simulink model "Compensated_FOC"  (R2023a)
settings: Solver=FixedStepDiscrete  StartTime=0.0  StopTime=SC.T  FixedStep=P.dt  RelTol=1e-3
PreLoadFcn:
  | d_ = fileparts(get_param(bdroot,'FileName')); addpath(d_, fullfile(d_, '..', 'Common')); clear d_; comp_foc_init;
values from neighbouring files (symbols this model uses):
  DECIM = 10    [comp_foc_init.m]
  P = bldc_params()    [comp_foc_init.m]
  TAB = struct()    [comp_foc_init.m]
  TAB_SHIFT = 0    [comp_foc_calib.mat]    (also in comp_foc_init.m; run_comp_foc.m = shv(bs))
  THETA_OFF = -1.57079632679    [comp_foc_calib.mat]    (also in comp_foc_init.m)
libraries: bldc_plant_lib x6, slpidlib x3, spspowerguiLib x1
settings Model: Creator=PC  LastModifiedBy=PC

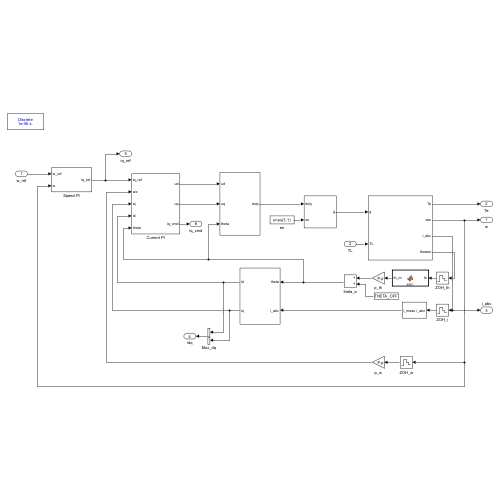
[thumbnail: Simulink's stored preview of the top-level diagram]
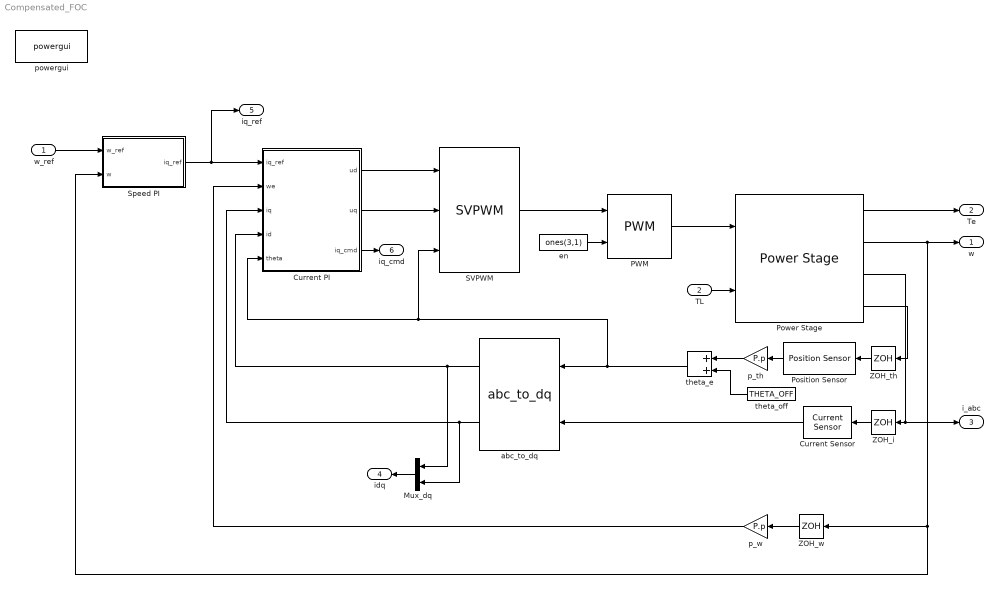
== system Compensated_FOC ==
  w_ref : Inport  Interpolate=off
  TL : Inport  Port=2  Interpolate=off
  Current PI : Subsystem
  Current Sensor : bldc_plant_lib/Current Sensor  Description=Phase-current sensors: i_meas = P.CS.M*(P.CS.gain.*i_abc + P.CS.off). Ideal by default (bldc_set_sensor).  SystemSampleTime=-1  VariantActivationTime=update diagram  Latency=0  AutoFrameSizeCalculation=off
  Mux_dq : Mux  Inputs=2
  PWM : bldc_plant_lib/PWM  SystemSampleTime=-1  VariantActivationTime=update diagram  Latency=0  AutoFrameSizeCalculation=off
  Position Sensor : bldc_plant_lib/Position Sensor  Description=Position sensor: quantized mechanical angle + mounting offset (P.ENC, bldc_set_encoder). Ideal by default.  SystemSampleTime=-1  VariantActivationTime=update diagram  Latency=0  AutoFrameSizeCalculation=off
      settings: LibrarySourceBlock=|
      | simulink/User-Defined
      | Functions/MATLAB Function
  Power Stage : bldc_plant_lib/Power Stage  SystemSampleTime=-1  VariantActivationTime=update diagram  Latency=0  AutoFrameSizeCalculation=off
  SVPWM : bldc_plant_lib/SVPWM  SystemSampleTime=-1  VariantActivationTime=update diagram  Latency=0  AutoFrameSizeCalculation=off
  Speed PI : Subsystem
  ZOH_i : ZeroOrderHold  SampleTime=P.Ts
  ZOH_th : ZeroOrderHold  SampleTime=P.Ts
  ZOH_w : ZeroOrderHold  SampleTime=P.Ts
  abc_to_dq : bldc_plant_lib/abc_to_dq  SystemSampleTime=-1  VariantActivationTime=update diagram  Latency=0  AutoFrameSizeCalculation=off
  en : Constant  Value=ones(3,1)
  p_th : Gain  Gain=P.p
  p_w : Gain  Gain=P.p
  powergui : spspowerguiLib/powergui  Priority=1  SimulationMode=Discrete  SampleTime=P.dt  frequency=60  Iterations=50  frequencyindice=0  Pbase=100e6  ErrMax=1e-4  UnitsV=kV  UnitsW=MW  buscounter=0  FunctionMessages=off  echomessages=off  EnableUseOfTLC=off  CurrentSourceSwitches=off  DisableSnubberDevices=off  DisableRonSwitches=off  DisableVfSwitches=off  DisplayEquations=off  AutomaticDiscreteSolvers=off  SolverType=Tustin/Backward Euler (TBE)  Interpol=off  ExternalGateDelay=off  methode=off  Ts=100  x0status=blocks  SPID=on  SwTol=0  HookPort=off  NonlinearTolerance=1e-4  nMaxIteration=100  ContinueOnMaxIteration=off  RestoreLinks=warning  ResistiveCurrentMeasurement=off  Frange=[0:2:500]  Ylog=off  Xlog=on  ShowGrid=off  save=off  variable=ZData  structure=0  ZoomFFT=off  StartTime=0.0  cycles=1  DisplayStyle=1  fundamental=60  FreqAxis=off  MaxFrequency=1000  frequencyindicesteady=1  RmsSteady=1  display=off
  theta_e : Sum
  theta_off : Constant  Value=THETA_OFF
  w : Outport  SampleTime=DECIM*P.dt
  Te : Outport  Port=2  SampleTime=DECIM*P.dt
  i_abc : Outport  Port=3  SampleTime=DECIM*P.dt
  idq : Outport  Port=4
  iq_ref : Outport  Port=5
  iq_cmd : Outport  Port=6
  wires:
  w_ref/1 -> Speed PI/1(w_ref)
  Speed PI/1(iq_ref) -> Current PI/1(iq_ref), iq_ref/1
  Current PI/1(ud) -> SVPWM/1
  Current PI/2(uq) -> SVPWM/2
  Current PI/3(iq_cmd) -> iq_cmd/1
  SVPWM/1 -> PWM/1
  en/1 -> PWM/2
  PWM/1 -> Power Stage/1
  TL/1 -> Power Stage/2
  Power Stage/1 -> Te/1
  Power Stage/2 -> ZOH_w/1, Speed PI/2(w), w/1
  Power Stage/3 -> ZOH_i/1, i_abc/1
  Power Stage/4 -> ZOH_th/1
  p_th/1 -> theta_e/1
  theta_off/1 -> theta_e/2
  theta_e/1 -> abc_to_dq/1, Current PI/5(theta), SVPWM/3
  abc_to_dq/1 -> Current PI/4(id), Mux_dq/1
  abc_to_dq/2 -> Current PI/3(iq), Mux_dq/2
  Mux_dq/1 -> idq/1
  ZOH_w/1 -> p_w/1
  p_w/1 -> Current PI/2(we)
  ZOH_i/1 -> Current Sensor/1
  Current Sensor/1 -> abc_to_dq/2
  ZOH_th/1 -> Position Sensor/1
  Position Sensor/1 -> p_th/1

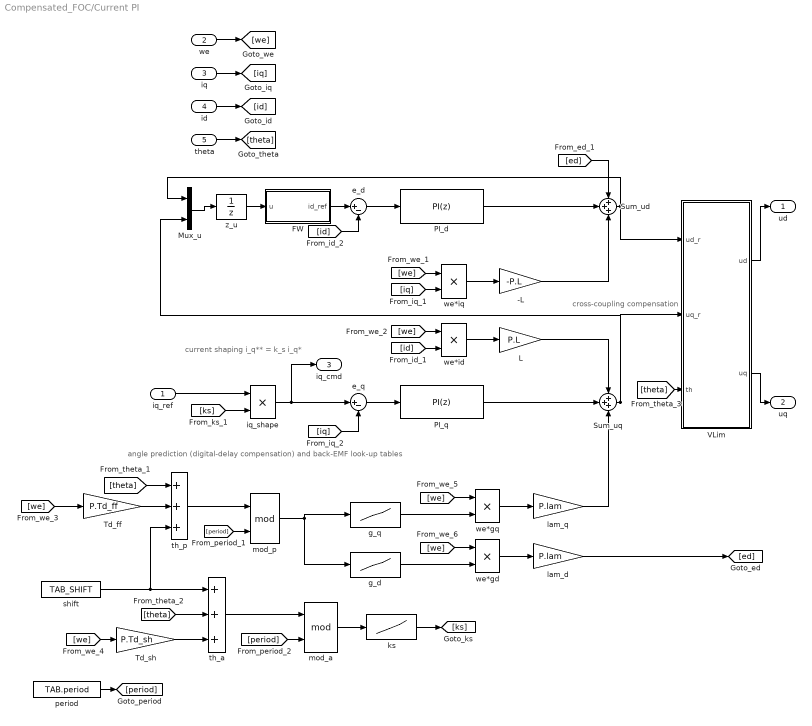
== system Compensated_FOC/Current PI ==
  note: cross-coupling compensation
  note: angle prediction (digital-delay compensation) and back-EMF look-up tables
  note: current shaping i_q** = k_s i_q*
  iq_ref : Inport
  we : Inport  Port=2
  iq : Inport  Port=3
  id : Inport  Port=4
  theta : Inport  Port=5
  -L : Gain  Gain=-P.L
  FW : MATLAB Function  TreatAsAtomicUnit=on  SystemSampleTime=P.Ts
  L : Gain  Gain=P.L
  Mux_u : Mux  Inputs=2
  PI_d : slpidlib/PID Controller  Controller=PI  Form=Parallel  TimeDomain=Discrete-time  UseExternalTs=off  SampleTime=P.Ts  IntegratorMethod=Forward Euler  FilterMethod=Forward Euler  ControllerParametersSource=internal  P=P.Kp_i  I=P.Ki_i  UseKiTs=off  D=0  N=100  UseFilter=on  TunerSelectOption=Transfer Function Based (PID Tuner App)  InitialConditionSource=internal  InitialConditionForIntegrator=0  InitialConditionForFilter=0  DifferentiatorICPrevScaledInput=0  ExternalReset=none  TrackingMode=off  Kt=1  LimitOutput=on  SatLimitsSource=internal  UpperSaturationLimit=P.Vm  LowerSaturationLimit=-P.Vm  LinearizeAsGain=off  AntiWindupMode=back-calculation  Kb=(P.Ki_i)/(P.Kp_i)  LimitIntegrator=off  UpperIntegratorSaturationLimit=inf  LowerIntegratorSaturationLimit=-inf  POutMin=[]  POutMax=[]  IOutMin=[]  IOutMax=[]  DOutMin=[]  DOutMax=[]  NOutMin=[]  NOutMax=[]  SumOutMin=[]  SumOutMax=[]  SaturationOutMin=[]  SaturationOutMax=[]  PParamMin=[]  PParamMax=[]  IParamMin=[]  IParamMax=[]  DParamMin=[]  DParamMax=[]  NParamMin=[]  NParamMax=[]  KbParamMin=[]  KbParamMax=[]  KtParamMin=[]  KtParamMax=[]  KbOutMin=[]  KbOutMax=[]  KtOutMin=[]  KtOutMax=[]  IntegratorOutMin=[]  IntegratorOutMax=[]  FilterOutMin=[]  FilterOutMax=[]  SumI1OutMin=[]  SumI1OutMax=[]  SumI2OutMin=[]  SumI2OutMax=[]  SumI3OutMin=[]  SumI3OutMax=[]  SumI4OutMin=[]  SumI4OutMax=[]  SumDOutMin=[]  SumDOutMax=[]  DifferentiatorOutMin=[]  DifferentiatorOutMax=[]  FilterDiffOutCoefMin=[]  FilterDiffOutCoefMax=[]  ReciprocalOutMin=[]  ReciprocalOutMax=[]  SumDenOutMin=[]  SumDenOutMax=[]  SumNumOutMin=[]  SumNumOutMax=[]  DivideOutMin=[]  DivideOutMax=[]  UdiffTsProdOutMin=[]  UdiffTsProdOutMax=[]  NTsProdOutMin=[]  NTsProdOutMax=[]  UintegralTsProdOutMin=[]  UintegralTsProdOutMax=[]  UngainTsProdOutMin=[]  UngainTsProdOutMax=[]  ClampingZeroOutDataTypeStr=Inherit: Inherit via back propagation  ClampingZeroOutMin=[]  ClampingZeroOutMax=[]  FilterDenConstantOutDataTypeStr=Inherit: Inherit via back propagation  FilterDenConstantOutMin=[]  FilterDenConstantOutMax=[]  PCopyOutDataTypeStr=Inherit: Inherit via back propagation  PCopyOutMin=[]  PCopyOutMax=[]  NCopyOutDataTypeStr=Inherit: Inherit via back propagation  NCopyOutMin=[]  NCopyOutMax=[]  IntegratorContinuousStateAttributes=''  IntegratorStateMustResolveToSignalObject=off  IntegratorRTWStateStorageClass=Auto  FilterContinuousStateAttributes=''  FilterStateMustResolveToSignalObject=off  FilterRTWStateStorageClass=Auto  ParallelPVariant=InternalParameters  IdealPVariant=Disabled  IVariant=InternalParameters  DVariant=Disabled  IntegratorVariant=Discrete  SatVariant=Enabled  AWVariant=BackCalculation  PCopyVariant=Disabled  TRVariant=Disabled  FdbkBlocksVariant=Forward  IdealPFdbkVariant=Disabled  SatFdbkVariant=Disabled  DerivativeFilterVariant=Disabled  NVariant=Disabled  NCopyVariant=Disabled_SignalSpec  FilterICVariant=Disabled  IntegratorICVariant=InternalICs  ExternalResetVariant=Disabled  TRSumVariant=Passthrough  SumFdbkVariant=Disabled  SumVariant=Sum_PI  TsampFilterVariant=InternalTs  TsampNgainVariant=Passthrough  TsampIntegralVariant=Disabled_SignalSpec  ExternalSaturationOutDataTypeStr=Inherit: Same as second input
      settings: LibrarySourceBlock=simulink/Discrete/Discrete PID Controller
  PI_q : slpidlib/PID Controller  Controller=PI  Form=Parallel  TimeDomain=Discrete-time  UseExternalTs=off  SampleTime=P.Ts  IntegratorMethod=Forward Euler  FilterMethod=Forward Euler  ControllerParametersSource=internal  P=P.Kp_i  I=P.Ki_i  UseKiTs=off  D=0  N=100  UseFilter=on  TunerSelectOption=Transfer Function Based (PID Tuner App)  InitialConditionSource=internal  InitialConditionForIntegrator=0  InitialConditionForFilter=0  DifferentiatorICPrevScaledInput=0  ExternalReset=none  TrackingMode=off  Kt=1  LimitOutput=on  SatLimitsSource=internal  UpperSaturationLimit=P.Vm  LowerSaturationLimit=-P.Vm  LinearizeAsGain=off  AntiWindupMode=back-calculation  Kb=(P.Ki_i)/(P.Kp_i)  LimitIntegrator=off  UpperIntegratorSaturationLimit=inf  LowerIntegratorSaturationLimit=-inf  POutMin=[]  POutMax=[]  IOutMin=[]  IOutMax=[]  DOutMin=[]  DOutMax=[]  NOutMin=[]  NOutMax=[]  SumOutMin=[]  SumOutMax=[]  SaturationOutMin=[]  SaturationOutMax=[]  PParamMin=[]  PParamMax=[]  IParamMin=[]  IParamMax=[]  DParamMin=[]  DParamMax=[]  NParamMin=[]  NParamMax=[]  KbParamMin=[]  KbParamMax=[]  KtParamMin=[]  KtParamMax=[]  KbOutMin=[]  KbOutMax=[]  KtOutMin=[]  KtOutMax=[]  IntegratorOutMin=[]  IntegratorOutMax=[]  FilterOutMin=[]  FilterOutMax=[]  SumI1OutMin=[]  SumI1OutMax=[]  SumI2OutMin=[]  SumI2OutMax=[]  SumI3OutMin=[]  SumI3OutMax=[]  SumI4OutMin=[]  SumI4OutMax=[]  SumDOutMin=[]  SumDOutMax=[]  DifferentiatorOutMin=[]  DifferentiatorOutMax=[]  FilterDiffOutCoefMin=[]  FilterDiffOutCoefMax=[]  ReciprocalOutMin=[]  ReciprocalOutMax=[]  SumDenOutMin=[]  SumDenOutMax=[]  SumNumOutMin=[]  SumNumOutMax=[]  DivideOutMin=[]  DivideOutMax=[]  UdiffTsProdOutMin=[]  UdiffTsProdOutMax=[]  NTsProdOutMin=[]  NTsProdOutMax=[]  UintegralTsProdOutMin=[]  UintegralTsProdOutMax=[]  UngainTsProdOutMin=[]  UngainTsProdOutMax=[]  ClampingZeroOutDataTypeStr=Inherit: Inherit via back propagation  ClampingZeroOutMin=[]  ClampingZeroOutMax=[]  FilterDenConstantOutDataTypeStr=Inherit: Inherit via back propagation  FilterDenConstantOutMin=[]  FilterDenConstantOutMax=[]  PCopyOutDataTypeStr=Inherit: Inherit via back propagation  PCopyOutMin=[]  PCopyOutMax=[]  NCopyOutDataTypeStr=Inherit: Inherit via back propagation  NCopyOutMin=[]  NCopyOutMax=[]  IntegratorContinuousStateAttributes=''  IntegratorStateMustResolveToSignalObject=off  IntegratorRTWStateStorageClass=Auto  FilterContinuousStateAttributes=''  FilterStateMustResolveToSignalObject=off  FilterRTWStateStorageClass=Auto  ParallelPVariant=InternalParameters  IdealPVariant=Disabled  IVariant=InternalParameters  DVariant=Disabled  IntegratorVariant=Discrete  SatVariant=Enabled  AWVariant=BackCalculation  PCopyVariant=Disabled  TRVariant=Disabled  FdbkBlocksVariant=Forward  IdealPFdbkVariant=Disabled  SatFdbkVariant=Disabled  DerivativeFilterVariant=Disabled  NVariant=Disabled  NCopyVariant=Disabled_SignalSpec  FilterICVariant=Disabled  IntegratorICVariant=InternalICs  ExternalResetVariant=Disabled  TRSumVariant=Passthrough  SumFdbkVariant=Disabled  SumVariant=Sum_PI  TsampFilterVariant=InternalTs  TsampNgainVariant=Passthrough  TsampIntegralVariant=Disabled_SignalSpec  ExternalSaturationOutDataTypeStr=Inherit: Same as second input
      settings: LibrarySourceBlock=simulink/Discrete/Discrete PID Controller
  Sum_ud : Sum  Inputs=+++
  Sum_uq : Sum  Inputs=+++
  Td_ff : Gain  Gain=P.Td_ff
  Td_sh : Gain  Gain=P.Td_sh
  VLim : MATLAB Function  TreatAsAtomicUnit=on  SystemSampleTime=P.Ts
  e_d : Sum  Inputs=|+-
  e_q : Sum  Inputs=|+-
  g_d : Lookup_n-D  NumberOfTableDimensions=1  BreakpointsForDimension1=TAB.th  Table=TAB.gd  ExtrapMethod=Clip  InternalRulePriority=Speed  RndMeth=Simplest
  g_q : Lookup_n-D  NumberOfTableDimensions=1  BreakpointsForDimension1=TAB.th  Table=TAB.gq  ExtrapMethod=Clip  InternalRulePriority=Speed  RndMeth=Simplest
  iq_shape : Product
  ks : Lookup_n-D  NumberOfTableDimensions=1  BreakpointsForDimension1=TAB.th  Table=TAB.ks  ExtrapMethod=Clip  InternalRulePriority=Speed  RndMeth=Simplest
  lam_d : Gain  Gain=P.lam
  lam_q : Gain  Gain=P.lam
  mod_a : Math  Operator=mod
  mod_p : Math  Operator=mod
  period : Constant  Value=TAB.period
  shift : Constant  Value=TAB_SHIFT
  th_a : Sum  Inputs=+++
  th_p : Sum  Inputs=+++
  we*gd : Product
  we*gq : Product
  we*id : Product
  we*iq : Product
  z_u : UnitDelay  InitialCondition=[0;0]  SampleTime=P.Ts
  ud : Outport
  uq : Outport  Port=2
  iq_cmd : Outport  Port=3
  wires:
  we/1 -> [we]
  [we] -> we*iq/1
  [we] -> we*id/1
  [we] -> Td_ff/1
  [we] -> Td_sh/1
  [we] -> we*gq/1
  [we] -> we*gd/1
  iq/1 -> [iq]
  [iq] -> we*iq/2
  [iq] -> e_q/2
  id/1 -> [id]
  [id] -> we*id/2
  [id] -> e_d/2
  theta/1 -> [theta]
  [theta] -> th_p/1
  [theta] -> th_a/2
  lam_d/1 -> [ed]
  [ed] -> Sum_ud/1
  period/1 -> [period]
  [period] -> mod_p/2
  [period] -> mod_a/2
  ks/1 -> [ks]
  [ks] -> iq_shape/2
  -L/1 -> Sum_ud/3
  L/1 -> Sum_uq/1
  PI_d/1 -> Sum_ud/2
  PI_q/1 -> Sum_uq/2
  Td_ff/1 -> th_p/2
  Td_sh/1 -> th_a/3
  e_d/1 -> PI_d/1
  e_q/1 -> PI_q/1
  g_d/1 -> we*gd/2
  g_q/1 -> we*gq/2
  iq_ref/1 -> iq_shape/1
  iq_shape/1 -> e_q/1, iq_cmd/1
  lam_q/1 -> Sum_uq/3
  mod_a/1 -> ks/1
  mod_p/1 -> g_d/1, g_q/1
  shift/1 -> th_p/3, th_a/1
  th_a/1 -> mod_a/1
  th_p/1 -> mod_p/1
  we*gd/1 -> lam_d/1
  we*gq/1 -> lam_q/1
  we*id/1 -> L/1
  we*iq/1 -> -L/1
  Sum_ud/1 -> VLim/1(ud_r), Mux_u/1
  Sum_uq/1 -> VLim/2(uq_r), Mux_u/2
  [theta] -> VLim/3(th)
  VLim/1(ud) -> ud/1
  VLim/2(uq) -> uq/1
  Mux_u/1 -> z_u/1
  z_u/1 -> FW/1(u)
  FW/1(id_ref) -> e_d/1

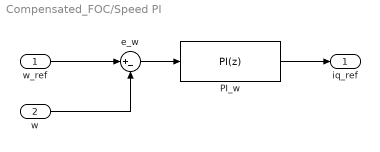
== system Compensated_FOC/Speed PI ==
  w_ref : Inport
  w : Inport  Port=2
  PI_w : slpidlib/PID Controller  Controller=PI  Form=Parallel  TimeDomain=Discrete-time  UseExternalTs=off  SampleTime=P.Tsw  IntegratorMethod=Forward Euler  FilterMethod=Forward Euler  ControllerParametersSource=internal  P=P.Kp_w_foc  I=P.Ki_w_foc  UseKiTs=off  D=0  N=100  UseFilter=on  TunerSelectOption=Transfer Function Based (PID Tuner App)  InitialConditionSource=internal  InitialConditionForIntegrator=0  InitialConditionForFilter=0  DifferentiatorICPrevScaledInput=0  ExternalReset=none  TrackingMode=off  Kt=1  LimitOutput=on  SatLimitsSource=internal  UpperSaturationLimit=P.Imax  LowerSaturationLimit=-P.Imax  LinearizeAsGain=off  AntiWindupMode=back-calculation  Kb=(P.Ki_w_foc)/(P.Kp_w_foc)  LimitIntegrator=off  UpperIntegratorSaturationLimit=inf  LowerIntegratorSaturationLimit=-inf  POutMin=[]  POutMax=[]  IOutMin=[]  IOutMax=[]  DOutMin=[]  DOutMax=[]  NOutMin=[]  NOutMax=[]  SumOutMin=[]  SumOutMax=[]  SaturationOutMin=[]  SaturationOutMax=[]  PParamMin=[]  PParamMax=[]  IParamMin=[]  IParamMax=[]  DParamMin=[]  DParamMax=[]  NParamMin=[]  NParamMax=[]  KbParamMin=[]  KbParamMax=[]  KtParamMin=[]  KtParamMax=[]  KbOutMin=[]  KbOutMax=[]  KtOutMin=[]  KtOutMax=[]  IntegratorOutMin=[]  IntegratorOutMax=[]  FilterOutMin=[]  FilterOutMax=[]  SumI1OutMin=[]  SumI1OutMax=[]  SumI2OutMin=[]  SumI2OutMax=[]  SumI3OutMin=[]  SumI3OutMax=[]  SumI4OutMin=[]  SumI4OutMax=[]  SumDOutMin=[]  SumDOutMax=[]  DifferentiatorOutMin=[]  DifferentiatorOutMax=[]  FilterDiffOutCoefMin=[]  FilterDiffOutCoefMax=[]  ReciprocalOutMin=[]  ReciprocalOutMax=[]  SumDenOutMin=[]  SumDenOutMax=[]  SumNumOutMin=[]  SumNumOutMax=[]  DivideOutMin=[]  DivideOutMax=[]  UdiffTsProdOutMin=[]  UdiffTsProdOutMax=[]  NTsProdOutMin=[]  NTsProdOutMax=[]  UintegralTsProdOutMin=[]  UintegralTsProdOutMax=[]  UngainTsProdOutMin=[]  UngainTsProdOutMax=[]  ClampingZeroOutDataTypeStr=Inherit: Inherit via back propagation  ClampingZeroOutMin=[]  ClampingZeroOutMax=[]  FilterDenConstantOutDataTypeStr=Inherit: Inherit via back propagation  FilterDenConstantOutMin=[]  FilterDenConstantOutMax=[]  PCopyOutDataTypeStr=Inherit: Inherit via back propagation  PCopyOutMin=[]  PCopyOutMax=[]  NCopyOutDataTypeStr=Inherit: Inherit via back propagation  NCopyOutMin=[]  NCopyOutMax=[]  IntegratorContinuousStateAttributes=''  IntegratorStateMustResolveToSignalObject=off  IntegratorRTWStateStorageClass=Auto  FilterContinuousStateAttributes=''  FilterStateMustResolveToSignalObject=off  FilterRTWStateStorageClass=Auto  ParallelPVariant=InternalParameters  IdealPVariant=Disabled  IVariant=InternalParameters  DVariant=Disabled  IntegratorVariant=Discrete  SatVariant=Enabled  AWVariant=BackCalculation  PCopyVariant=Disabled  TRVariant=Disabled  FdbkBlocksVariant=Forward  IdealPFdbkVariant=Disabled  SatFdbkVariant=Disabled  DerivativeFilterVariant=Disabled  NVariant=Disabled  NCopyVariant=Disabled_SignalSpec  FilterICVariant=Disabled  IntegratorICVariant=InternalICs  ExternalResetVariant=Disabled  TRSumVariant=Passthrough  SumFdbkVariant=Disabled  SumVariant=Sum_PI  TsampFilterVariant=InternalTs  TsampNgainVariant=Passthrough  TsampIntegralVariant=Disabled_SignalSpec  ExternalSaturationOutDataTypeStr=Inherit: Same as second input
      settings: LibrarySourceBlock=simulink/Discrete/Discrete PID Controller
  e_w : Sum  Inputs=|+-
  iq_ref : Outport
  wires:
  PI_w/1 -> iq_ref/1
  e_w/1 -> PI_w/1
  w/1 -> e_w/2
  w_ref/1 -> e_w/1

== matlab function Compensated_FOC/Current PI/FW ==
  data: u input; id_ref output; P parameter
function id_ref = FW(u, P)
% field weakening by voltage feedback (P.FW, Common/bldc_params.m)
% u = [u_d; u_q] requested before the limiter, delayed by one sample
persistent x
if isempty(x), x = 0; end
id_ref = 0;
if P.FW.on
    id_ref = x;
    x = x + P.Ts*P.FW.Ki*(P.FW.k*P.Vm - sqrt(u(1)^2 + u(2)^2));
    x = min(0, max(-P.FW.Idmax, x));
end

== matlab function Compensated_FOC/Current PI/VLim ==
  data: ud_r input; ud output; uq_r input; th input; uq output; P parameter
function [ud, uq] = VLim(ud_r, uq_r, th, P)
% voltage limiter, strategy P.vlim (see Common/bldc_vlim.m)
[ud, uq] = bldc_vlim(ud_r, uq_r, th, P);
